simulink library "sf_aircraft_sensor_lib"  (R2025b)
settings: Solver=VariableStepAuto  StartTime=0.0  StopTime=10.0  RelTol=1e-3
undefined symbols (not defined in the file or in its folder): DEBOUNCE, MAXDELTA, MAXDIFF, MAXVAL, MINVAL, N
settings Model: Creator=The MathWorks, Inc.  LastModifiedBy=The MathWorks, Inc.

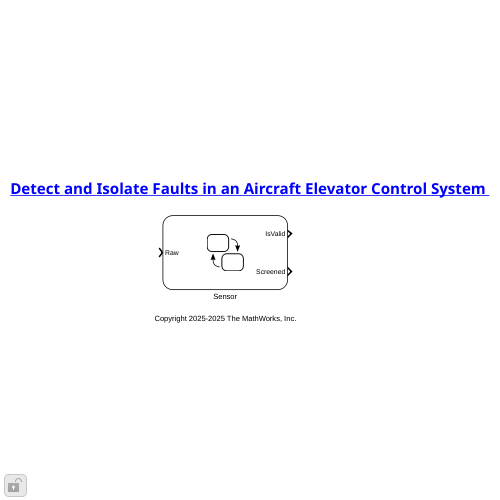
[thumbnail: Simulink's stored preview of the top-level diagram]
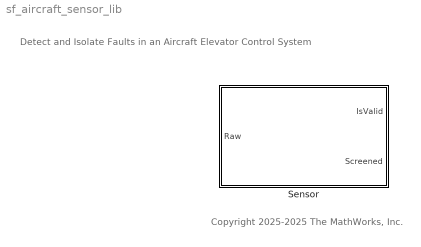
== system sf_aircraft_sensor_lib ==
  note: Copyright 2025-2025 The MathWorks, Inc.
  note: Detect and Isolate Faults in an Aircraft Elevator Control System
  Sensor : Stateflow chart  TreatAsAtomicUnit=on

== stateflow chart sf_aircraft_sensor_lib/Sensor ==
  state Valid
    en, du:
    Screened = Raw(N);
    RawPrevious = Raw(N);
    IsValid = 1;
  state Invalid
    en, du:
    Screened = NaN;
    RawPrevious = Raw(N);
    IsValid = 0;
  (default) -> Valid
  Valid -> (junction 19)
  (junction 19) -> Invalid [order 1] : %Change to outside the valid bounce for greater than DEBOUNCE sec
      | [duration(Raw(N) > MAXVAL || Raw(N) < MINVAL,sec) > DEBOUNCE]
  (junction 19) -> (junction 21) [order 2]
  (junction 21) -> Invalid [order 1] : %Change larger than allowed delta for larger than DEBOUNCE sec
      | [duration(abs(Raw(N)-(RawPrevious)) > MAXDELTA,sec) > DEBOUNCE]
  (junction 21) -> (junction 23) [order 2]
  (junction 23) -> Invalid : %One sensor is different than the mean by more than MAXDIFF
      | [abs(Raw(N)-mean(Raw)) > MAXDIFF]
  Invalid -> Valid : %Sensor reading has returned to valid values for longer than DEBOUNCE sec
      | [duration(Raw(N) < MAXVAL && Raw(N) > MINVAL, sec) > DEBOUNCE && ...
      | duration(abs(Raw(N)-(RawPrevious)) < MAXDELTA,sec) > DEBOUNCE && ...
      | abs(Raw(N)-mean(Raw)) < MAXDIFF]
  data: Raw input double size=3; IsValid output uint8 size=1 =1; Screened output double size=1 =0; DEBOUNCE parameter; MAXDELTA parameter; MAXDIFF parameter; MAXVAL parameter; MINVAL parameter; N parameter; RawPrevious local double size=1 =0
